simulink library "Tire_MFEval"  (R2026a)
settings: Solver=VariableStepAuto
undefined symbols (not defined in the file): Tire, Visual
libraries: nesl_utility x11, sm_lib x3, mfeval_LIB x1, Tire_Utilities x1, TireBody_Systems x1
Description:
  | Component of Simscape Vehicle Templates Library
  | 
  | Copyright 2018-2024 The MathWorks, Inc.
settings Model: Creator=smiller  LastModifiedBy=andrei

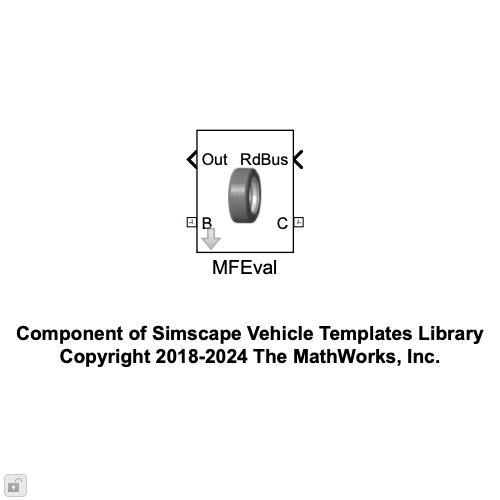
[thumbnail: Simulink's stored preview of the top-level diagram]
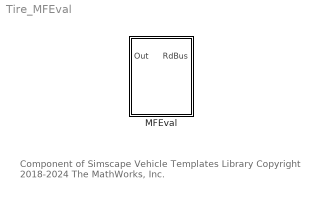
== system Tire_MFEval ==
  note: Component of Simscape Vehicle Templates Library
      | Copyright 2018-2024 The MathWorks, Inc.
  MFEval : Subsystem  VariantControl=MFEval  mask(MFeval Tire){tir_file=Tire.tirFile.Value, tir_side=2 right, tir_dynamics=Tire.Dynamics.Value, tir_mode=Tire.Mode.Value, TireBody=Tire.TireBody, popup_leftRight=Right, clr_tyre=Visual.Tire.clr, opc_tyre=Visual.Tire.opc, clr_rim=Visual.Rim.clrVisual.Rim.clr, opc_rim=Visual.Rim.opc}
      mask prompts: tir_file "TIR File (String variable)"; tir_side "Tyre side     :"; tir_dynamics "Dynamics"; tir_mode "Mode"; TireBody "Tire Body (structure)"; popup_leftRight "Left/Right"
      mask help: Models tire using MFeval tire software.
      mask init:
      | curblk = gcb;
      | tir_file = strrep(tir_file,"''","'");
      | temptirparams = mfeval.readTIR(eval(tir_file));
      | tire_radius = temptirparams.UNLOADED_RADIUS;
      | tire_width  = temptirparams.WIDTH;
      | rim_radius  = temptirparams.RIM_RADIUS;
      | rim_width   = tire_width*0.1;
      | tyre_mass   = temptirparams.MASS1;
      | %if(isnan(tire_mass))
      | %    tire_mass = 15;
      | %end
      | TireStruct = temptirparams;
      | tyre_Ixx   = temptirparams.IXX;
      | tyre_Iyy   = temptirparams.IYY;
      | 
      | tire_kvert  = temptirparams.VERTICAL_STIFFNESS;
      | tire_bvert  = temptirparams.VERTICAL_DAMPING;
      | 
      | %set_param([gcb '/CPI tyre'],'userSide',tir_sie);
      | set_param([gcb '/CPI tyre'],'userDynamics',tir_dynamics);
      | set_param([gcb '/CPI tyre'],'userUseMode',tir_mode);
      | 
      | if(popup_leftRight == 1)
      |     set_param([gcb '/Tire Body'],'popup_leftRight','Left');
      | elseif(popup_leftRight == 2)
      |     set_param([gcb '/Tire Body'],'popup_leftRight','Right');
      | end
      mask TypeOptions tir_side: CPI tyre/userSide
      mask TypeOptions popup_leftRight: Left | Right
      mask TypeOptions clr_tyre: Tire Body/clr_tyre
      mask TypeOptions opc_tyre: Tire Body/opc_tyre
      mask TypeOptions clr_rim: Tire Body/clr_rim
      mask TypeOptions opc_rim: Tire Body/opc_rim
      mask DialogControl cont_tire_mfeval Prompt: Tire
      mask DialogControl cont_vis Prompt: Visualization
      mask DialogControl text_vis_clr Prompt: Color [RGB]
      mask DialogControl text_vis_opc Prompt: Opacity (0-1)
      mask DialogControl text_tyre Prompt: Tyre
      mask DialogControl text_rim Prompt: Rim
      mask Display: image('sm_car_vehicle_tire_mfeval_IMAGE.png');

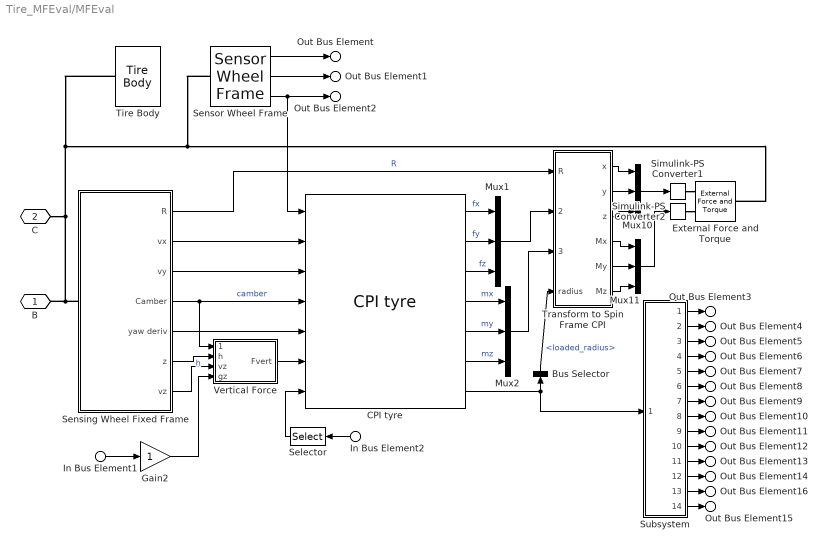
== system Tire_MFEval/MFEval ==
  In Bus Element1 : Inport  PortName=RdBus  Element=gz
  In Bus Element2 : Inport  PortName=RdBus  Element=TyreScaling
  Bus Selector : BusSelector  OutputSignals=loaded_radius
  CPI tyre : mfeval_LIB/CPI tyre  Description=Magic Formula 6.1.2 tyre model including relaxation length and transient calculations  userParameterSource=TireStruct  userSide=2 right  userDynamics=3 non-linear transients  userUseMode=1 combined  enablePressure=off  userPressure=0.5
      settings: SourceProductName=MFeval Library
  External Force and Torque : sm_lib/Forces and Torques/External Force and Torque  EnableForceX=off  EnableForceY=off  EnableForceZ=off  EnableForce=on  ForceResolutionFrame=AttachedFrame  EnableTorqueX=off  EnableTorqueY=off  EnableTorqueZ=off  EnableTorque=on  TorqueResolutionFrame=AttachedFrame
  Gain2 : Gain
  Mux{1..2,10..11} (4 alike) : Mux  Inputs=3
  Selector : Selector  InputPortWidth=7  IndexOptions=Index vector (dialog)  Indices=[1 3]  OutputSizes=1
  Sensing Wheel Fixed Frame : Subsystem
  Sensor Wheel Frame : Tire_Utilities/Sensor Wheel Frame  SystemSampleTime=-1  VariantActivationTime=update diagram  EmptyChoice=off  PassThrough=off  PassThroughVariantControl=(default)  EmptyChoiceVariantControl=(default)  AllowFlexibleInterface=on  Latency=0  AutoFrameSizeCalculation=off
  Simulink-PS Converter1 : nesl_utility/Simulink-PS Converter  PhysicalDomain=network_engine_domain  SubClassName=ps_input  LeftPortType=input  RightPortType=output  PseudoPeriodic=off  Frequencies=[]  NoiseDistribution=none  NoiseParameters=[]  Unit=N  AffineConversion=off  FilteringAndDerivatives=provide  SimscapeFilterOrder=1  InputFilterTimeConstant=0.001  UdotUserProvided=0
  Simulink-PS Converter2 : nesl_utility/Simulink-PS Converter  PhysicalDomain=network_engine_domain  SubClassName=ps_input  LeftPortType=input  RightPortType=output  PseudoPeriodic=off  Frequencies=[]  NoiseDistribution=none  NoiseParameters=[]  Unit=N*m  AffineConversion=off  FilteringAndDerivatives=provide  SimscapeFilterOrder=1  InputFilterTimeConstant=0.001  UdotUserProvided=0
  Subsystem : Subsystem
  Tire Body : TireBody_Systems/Tire Body  LabelModeActiveChoice=Parameterized  popup_leftRight=Left  TireBody=TireBody  VariantLabel=TireBody.class.Value
      settings: AttributesFormatString=%<LabelModeActiveChoice>
  Transform to Spin Frame CPI : Subsystem
  Vertical Force : Subsystem
  B : PMIOPort  Side=Right
  C : PMIOPort  Port=2  Side=Left
  Out Bus Element : Outport  VectorParamsAs1DForOutWhenUnconnected=off  PortName=Out  Element=qxyz
  Out Bus Element1 : Outport  VectorParamsAs1DForOutWhenUnconnected=off  PortName=Out  Element=xyz
  Out Bus Element2 : Outport  VectorParamsAs1DForOutWhenUnconnected=off  PortName=Out  Element=n
  Out Bus Element3 : Outport  VectorParamsAs1DForOutWhenUnconnected=off  PortName=Out  Element=Fx
  Out Bus Element4 : Outport  VectorParamsAs1DForOutWhenUnconnected=off  PortName=Out  Element=Fy
  Out Bus Element5 : Outport  VectorParamsAs1DForOutWhenUnconnected=off  PortName=Out  Element=Fz
  Out Bus Element6 : Outport  VectorParamsAs1DForOutWhenUnconnected=off  PortName=Out  Element=Mx
  Out Bus Element7 : Outport  VectorParamsAs1DForOutWhenUnconnected=off  PortName=Out  Element=My
  Out Bus Element8 : Outport  VectorParamsAs1DForOutWhenUnconnected=off  PortName=Out  Element=Mz
  Out Bus Element9 : Outport  VectorParamsAs1DForOutWhenUnconnected=off  PortName=Out  Element=rSlip
  Out Bus Element10 : Outport  VectorParamsAs1DForOutWhenUnconnected=off  PortName=Out  Element=aSlip
  Out Bus Element11 : Outport  VectorParamsAs1DForOutWhenUnconnected=off  PortName=Out  Element=aCamber
  Out Bus Element12 : Outport  VectorParamsAs1DForOutWhenUnconnected=off  PortName=Out  Element=vx
  Out Bus Element13 : Outport  VectorParamsAs1DForOutWhenUnconnected=off  PortName=Out  Element=rMuX
  Out Bus Element14 : Outport  VectorParamsAs1DForOutWhenUnconnected=off  PortName=Out  Element=rMuY
  Out Bus Element15 : Outport  VectorParamsAs1DForOutWhenUnconnected=off  PortName=Out  Element=r_eff
  Out Bus Element16 : Outport  VectorParamsAs1DForOutWhenUnconnected=off  PortName=Out  Element=r_l
  wires:
  Bus Selector/1 -> Transform to Spin Frame CPI/4(radius)  "<loaded_radius>"
  Sensor Wheel Frame/3 -> CPI tyre/1, Out Bus Element2/1
  Sensor Wheel Frame/2 -> Out Bus Element1/1
  Sensor Wheel Frame/1 -> Out Bus Element/1
  Mux1/1 -> Transform to Spin Frame CPI/2(Fcontact)
  Mux2/1 -> Transform to Spin Frame CPI/3(MContact)
  Mux10/1 -> Simulink-PS Converter1/1
  Transform to Spin Frame CPI/2(y) -> Mux10/2
  Transform to Spin Frame CPI/3(z) -> Mux10/3
  Transform to Spin Frame CPI/5(My) -> Mux11/2
  Transform to Spin Frame CPI/4(Mx) -> Mux11/1
  Transform to Spin Frame CPI/6(Mz) -> Mux11/3
  Transform to Spin Frame CPI/1(x) -> Mux10/1
  Mux11/1 -> Simulink-PS Converter2/1
  Gain2/1 -> Vertical Force/4(gz)
  Sensing Wheel Fixed Frame/7(vz) -> Vertical Force/3(vz)
  Sensing Wheel Fixed Frame/6(z) -> Vertical Force/2(h)  "h"
  Sensing Wheel Fixed Frame/4(Camber) -> Vertical Force/1(camber), CPI tyre/4  "camber"
  Sensing Wheel Fixed Frame/2(vx) -> CPI tyre/2
  CPI tyre/4 -> Mux2/1  "mx"
  CPI tyre/2 -> Mux1/2  "fy"
  CPI tyre/5 -> Mux2/2  "my"
  CPI tyre/6 -> Mux2/3  "mz"
  CPI tyre/3 -> Mux1/3  "fz"
  CPI tyre/1 -> Mux1/1  "fx"
  Vertical Force/1(Fvert) -> CPI tyre/6
  Sensing Wheel Fixed Frame/3(vy) -> CPI tyre/3
  Sensing Wheel Fixed Frame/5(yaw deriv) -> CPI tyre/5
  Sensing Wheel Fixed Frame/1(R) -> Transform to Spin Frame CPI/1(R)  "R"
  In Bus Element1/1 -> Gain2/1
  CPI tyre/7 -> Bus Selector/1, Subsystem/1(In1)
  Subsystem/1(<Fx>) -> Out Bus Element3/1
  Subsystem/2(<Fy>) -> Out Bus Element4/1
  Subsystem/3(<Fz>) -> Out Bus Element5/1
  Subsystem/4(<Mx>) -> Out Bus Element6/1
  Subsystem/5(<My>) -> Out Bus Element7/1
  Subsystem/6(<Mz>) -> Out Bus Element8/1
  Subsystem/7(<longitudinal_slip>) -> Out Bus Element9/1
  Subsystem/8(<side_slip_angle>) -> Out Bus Element10/1
  Subsystem/9(<inclination_angle>) -> Out Bus Element11/1
  Subsystem/10(<Vx>) -> Out Bus Element12/1
  Subsystem/11(<mu_x>) -> Out Bus Element13/1
  Subsystem/12(<mu_y>) -> Out Bus Element14/1
  In Bus Element2/1 -> Selector/1
  Selector/1 -> CPI tyre/7
  Subsystem/13(<r_l>) -> Out Bus Element16/1
  Subsystem/14(<r_eff>) -> Out Bus Element15/1
  connections:
  Simulink-PS Converter1/RConn1 -- External Force and Torque/LConn1
  Simulink-PS Converter2/RConn1 -- External Force and Torque/LConn2
  B/RConn1 -- Sensing Wheel Fixed Frame/LConn1 -- External Force and Torque/RConn1 -- Sensor Wheel Frame/LConn1 -- Tire Body/LConn1 -- C/RConn1

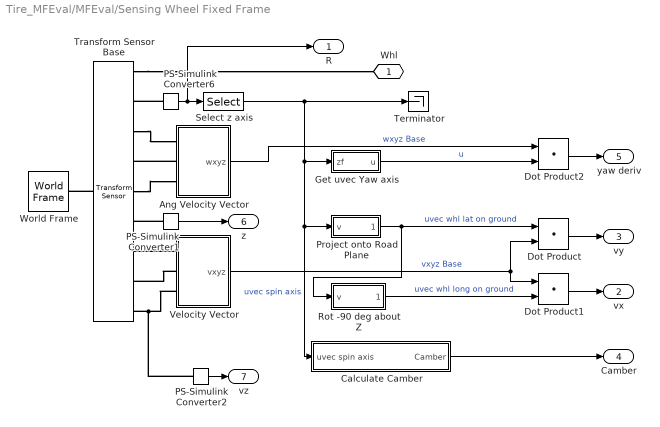
== system Tire_MFEval/MFEval/Sensing Wheel Fixed Frame ==
  Ang Velocity Vector : Subsystem
  Calculate Camber : Subsystem
  Dot Product : DotProduct  OutDataTypeStr=Inherit: Inherit via internal rule
  Dot Product1 : DotProduct  OutDataTypeStr=Inherit: Inherit via internal rule
  Dot Product2 : DotProduct  OutDataTypeStr=Inherit: Inherit via internal rule
  Get uvec Yaw axis : Subsystem
  PS-Simulink Converter1 : nesl_utility/PS-Simulink Converter  PhysicalDomain=network_engine_domain  SubClassName=ps_output  LeftPortType=input  RightPortType=output  PseudoPeriodic=off  Frequencies=[]  VectorFormat=1-D array  Unit=1  AffineConversion=off
  PS-Simulink Converter2 : nesl_utility/PS-Simulink Converter  PhysicalDomain=network_engine_domain  SubClassName=ps_output  LeftPortType=input  RightPortType=output  PseudoPeriodic=off  Frequencies=[]  VectorFormat=1-D array  Unit=1  AffineConversion=off
  PS-Simulink Converter6 : nesl_utility/PS-Simulink Converter  PhysicalDomain=network_engine_domain  SubClassName=ps_output  LeftPortType=input  RightPortType=output  PseudoPeriodic=off  Frequencies=[]  VectorFormat=1-D array  Unit=1  AffineConversion=off
  Project onto Road Plane : Subsystem
  Rot -90 deg about Z : Subsystem
  Select z axis : Selector  NumberOfDimensions=2  InputPortWidth=2  IndexOptions=Index vector (dialog),Index vector (dialog)  Indices=[1 2 3],3  OutputSizes=1,1
  Terminator : Terminator
  Transform Sensor Base : sm_lib/Frames and Transforms/Transform Sensor  MeasurementFrame=Base  RotationSequence=XYX  SenseAngle=off  SenseAxis=off  SenseQ=off  SenseR=on  SenseRotationSequence=off  SenseOmegaX=on  SenseOmegaY=on  SenseOmegaZ=on  SenseOmega=off  SenseQDot=off  SenseRDot=off  SenseRotationSequenceDot=off  SenseAlphaX=off  SenseAlphaY=off  SenseAlphaZ=off  SenseAlpha=off  SenseQDDot=off  SenseRDDot=off  SenseX=off  SenseY=off  SenseZ=on  SenseXYZ=off  SenseRad=off  SenseAzim=off  SenseDist=off  SenseInc=off  SenseXDot=on  SenseYDot=on  SenseZDot=on  SenseXYZDot=off  SenseRadDot=off  SenseAzimDot=off  SenseDistDot=off  SenseIncDot=off  SenseXDDot=off  SenseYDDot=off  SenseZDDot=off  SenseXYZDDot=off  SenseRadDDot=off  SenseAzimDDot=off  SenseDistDDot=off  SenseIncDDot=off
  Velocity Vector : Subsystem
  World Frame : sm_lib/Frames and Transforms/World Frame
  Whl : PMIOPort  Side=Left
  R : Outport  VectorParamsAs1DForOutWhenUnconnected=off
  vx : Outport  Port=2  VectorParamsAs1DForOutWhenUnconnected=off
  vy : Outport  Port=3  VectorParamsAs1DForOutWhenUnconnected=off
  Camber : Outport  Port=4  VectorParamsAs1DForOutWhenUnconnected=off
  yaw deriv : Outport  Port=5  VectorParamsAs1DForOutWhenUnconnected=off
  z : Outport  Port=6  VectorParamsAs1DForOutWhenUnconnected=off
  vz : Outport  Port=7  VectorParamsAs1DForOutWhenUnconnected=off
  wires:
  PS-Simulink Converter2/1 -> vz/1
  PS-Simulink Converter6/1 -> Select z axis/1, R/1
  Select z axis/1 -> Get uvec Yaw axis/1(zf), Calculate Camber/1(uvec spin axis), Project onto Road Plane/1(v), Terminator/1  "uvec spin axis"
  Rot -90 deg about Z/1(v rot -z) -> Dot Product1/2  "uvec whl long on ground"
  Velocity Vector/1(vxyz) -> Dot Product/2, Dot Product1/1  "vxyz Base"
  Get uvec Yaw axis/1(u) -> Dot Product2/2  "u"
  Ang Velocity Vector/1(wxyz) -> Dot Product2/1  "wxyz Base"
  Dot Product2/1 -> yaw deriv/1
  Project onto Road Plane/1(v proj) -> Rot -90 deg about Z/1(v), Dot Product/1  "uvec whl lat on ground"
  Dot Product/1 -> vy/1
  Dot Product1/1 -> vx/1
  PS-Simulink Converter1/1 -> z/1
  Calculate Camber/1(Camber) -> Camber/1
  connections:
  Transform Sensor Base/RConn1 -- Whl/RConn1
  PS-Simulink Converter6/LConn1 -- Transform Sensor Base/RConn2
  Transform Sensor Base/LConn1 -- World Frame/RConn1
  Transform Sensor Base/RConn3 -- Ang Velocity Vector/LConn1
  Ang Velocity Vector/LConn2 -- Transform Sensor Base/RConn4
  Transform Sensor Base/RConn5 -- Ang Velocity Vector/LConn3
  Velocity Vector/LConn1 -- Transform Sensor Base/RConn7
  Velocity Vector/LConn2 -- Transform Sensor Base/RConn8
  PS-Simulink Converter2/LConn1 -- Transform Sensor Base/RConn9 -- Velocity Vector/LConn3
  PS-Simulink Converter1/LConn1 -- Transform Sensor Base/RConn6

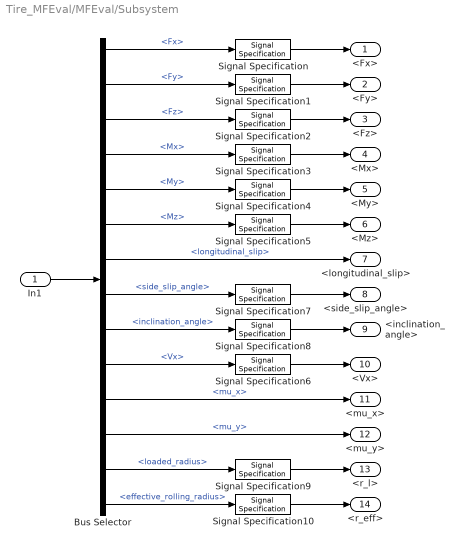
== system Tire_MFEval/MFEval/Subsystem ==
  In1 : Inport
  Bus Selector : BusSelector  OutputSignals=Fx,Fy,Fz,Mx,My,Mz,longitudinal_slip,side_slip_angle,inclination_angle,Vx,mu_x,mu_y,loaded_radius,effective_rolling_radius
  Signal Specification : SignalSpecification  Unit=N
  Signal Specification1 : SignalSpecification  Unit=N
  Signal Specification10 : SignalSpecification  Unit=m
  Signal Specification2 : SignalSpecification  Unit=N
  Signal Specification3 : SignalSpecification  Unit=N*m
  Signal Specification4 : SignalSpecification  Unit=N*m
  Signal Specification5 : SignalSpecification  Unit=N*m
  Signal Specification6 : SignalSpecification  Unit=m/s
  Signal Specification7 : SignalSpecification  Unit=rad
  Signal Specification8 : SignalSpecification  Unit=rad
  Signal Specification9 : SignalSpecification  Unit=m
  <Fx> : Outport  VectorParamsAs1DForOutWhenUnconnected=off
  <Fy> : Outport  Port=2  VectorParamsAs1DForOutWhenUnconnected=off
  <Fz> : Outport  Port=3  VectorParamsAs1DForOutWhenUnconnected=off
  <Mx> : Outport  Port=4  VectorParamsAs1DForOutWhenUnconnected=off
  <My> : Outport  Port=5  VectorParamsAs1DForOutWhenUnconnected=off
  <Mz> : Outport  Port=6  VectorParamsAs1DForOutWhenUnconnected=off
  <longitudinal_slip> : Outport  Port=7  VectorParamsAs1DForOutWhenUnconnected=off
  <side_slip_angle> : Outport  Port=8  VectorParamsAs1DForOutWhenUnconnected=off
  <inclination_angle> : Outport  Port=9  VectorParamsAs1DForOutWhenUnconnected=off
  <Vx> : Outport  Port=10  VectorParamsAs1DForOutWhenUnconnected=off
  <mu_x> : Outport  Port=11  VectorParamsAs1DForOutWhenUnconnected=off
  <mu_y> : Outport  Port=12  VectorParamsAs1DForOutWhenUnconnected=off
  <r_l> : Outport  Port=13  VectorParamsAs1DForOutWhenUnconnected=off
  <r_eff> : Outport  Port=14  VectorParamsAs1DForOutWhenUnconnected=off
  wires:
  Bus Selector/9 -> Signal Specification8/1  "<inclination_angle>"
  Bus Selector/10 -> Signal Specification6/1  "<Vx>"
  Bus Selector/2 -> Signal Specification1/1  "<Fy>"
  Bus Selector/4 -> Signal Specification3/1  "<Mx>"
  Bus Selector/3 -> Signal Specification2/1  "<Fz>"
  Bus Selector/11 -> <mu_x>/1  "<mu_x>"
  Bus Selector/6 -> Signal Specification5/1  "<Mz>"
  Bus Selector/1 -> Signal Specification/1  "<Fx>"
  Bus Selector/8 -> Signal Specification7/1  "<side_slip_angle>"
  Bus Selector/5 -> Signal Specification4/1  "<My>"
  Bus Selector/7 -> <longitudinal_slip>/1  "<longitudinal_slip>"
  Bus Selector/12 -> <mu_y>/1  "<mu_y>"
  In1/1 -> Bus Selector/1
  Signal Specification/1 -> <Fx>/1
  Signal Specification1/1 -> <Fy>/1
  Signal Specification2/1 -> <Fz>/1
  Signal Specification3/1 -> <Mx>/1
  Signal Specification4/1 -> <My>/1
  Signal Specification5/1 -> <Mz>/1
  Signal Specification6/1 -> <Vx>/1
  Signal Specification7/1 -> <side_slip_angle>/1
  Signal Specification8/1 -> <inclination_angle>/1
  Bus Selector/13 -> Signal Specification9/1  "<loaded_radius>"
  Bus Selector/14 -> Signal Specification10/1  "<effective_rolling_radius>"
  Signal Specification9/1 -> <r_l>/1
  Signal Specification10/1 -> <r_eff>/1

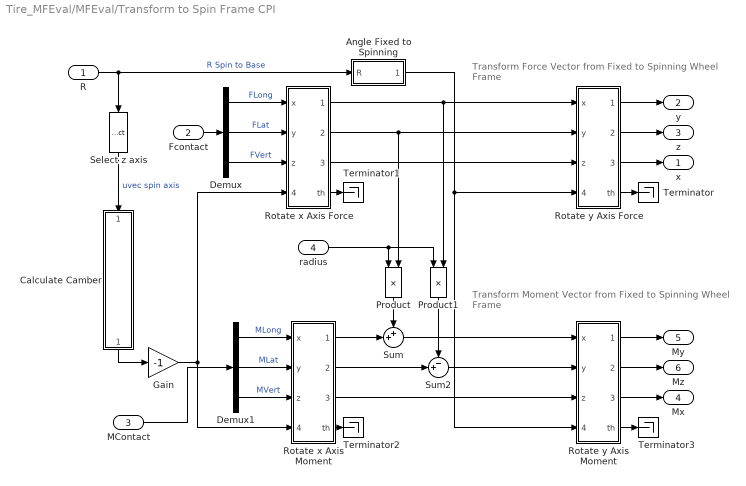
== system Tire_MFEval/MFEval/Transform to Spin Frame CPI ==
  note: Transform Moment Vector from Fixed
      | to Spinning Wheel Frame
  note: Transform Force Vector from Fixed
      | to Spinning Wheel Frame
  R : Inport
  Fcontact : Inport  Port=2
  MContact : Inport  Port=3
  radius : Inport  Port=4
  Angle Fixed to Spinning : Subsystem
  Calculate Camber : Subsystem
  Demux : Demux  Outputs=3
  Demux1 : Demux  Outputs=3
  Gain : Gain  Gain=-1
  Product : Product
  Product1 : Product
  Rotate x Axis Force : Subsystem
  Rotate x Axis Moment : Subsystem
  Rotate y Axis Force : Subsystem
  Rotate y Axis Moment : Subsystem
  Select z axis : Selector  NumberOfDimensions=2  InputPortWidth=2  IndexOptions=Index vector (dialog),Index vector (dialog)  Indices=[1 2 3],3  OutputSizes=1,1
  Sum : Sum  Inputs=++|
  Sum2 : Sum  Inputs=-+|
  Terminator{,1..3} (4 alike) : Terminator
  x : Outport  VectorParamsAs1DForOutWhenUnconnected=off
  y : Outport  Port=2  VectorParamsAs1DForOutWhenUnconnected=off
  z : Outport  Port=3  VectorParamsAs1DForOutWhenUnconnected=off
  Mx : Outport  Port=4  VectorParamsAs1DForOutWhenUnconnected=off
  My : Outport  Port=5  VectorParamsAs1DForOutWhenUnconnected=off
  Mz : Outport  Port=6  VectorParamsAs1DForOutWhenUnconnected=off
  wires:
  R/1 -> Select z axis/1, Angle Fixed to Spinning/1(R)  "R Spin to Base"
  Angle Fixed to Spinning/1(rotang) -> Rotate y Axis Moment/4(theta), Rotate y Axis Force/4(theta)
  Rotate y Axis Moment/1(x rot) -> My/1
  Rotate y Axis Moment/2(y rot) -> Mz/1
  Rotate x Axis Moment/1(x rot) -> Sum/2
  Rotate x Axis Force/1(x rot) -> Product1/2, Rotate y Axis Force/1(x)
  Rotate y Axis Force/1(x rot) -> y/1
  Rotate y Axis Force/2(y rot) -> z/1
  Select z axis/1 -> Calculate Camber/1(uvec spin axis)  "uvec spin axis"
  Demux/1 -> Rotate x Axis Force/1(x)  "FLong"
  Demux/3 -> Rotate x Axis Force/3(z)  "FVert"
  Calculate Camber/1(Camber) -> Gain/1
  Demux1/3 -> Rotate x Axis Moment/3(z)  "MVert"
  Demux1/1 -> Rotate x Axis Moment/1(x)  "MLong"
  Demux1/2 -> Rotate x Axis Moment/2(y)  "MLat"
  Product/1 -> Sum/1
  radius/1 -> Product1/1, Product/1
  Rotate x Axis Force/3(z rot) -> Rotate y Axis Force/3(z)
  Product1/1 -> Sum2/1
  Demux/2 -> Rotate x Axis Force/2(y)  "FLat"
  Rotate x Axis Force/2(y rot) -> Rotate y Axis Force/2(y), Product/2
  Rotate y Axis Force/3(z rot) -> x/1
  Rotate y Axis Force/4(th) -> Terminator/1
  Rotate x Axis Force/4(th) -> Terminator1/1
  Rotate x Axis Moment/2(y rot) -> Sum2/2
  Rotate x Axis Moment/4(th) -> Terminator2/1
  Rotate y Axis Moment/3(z rot) -> Mx/1
  Rotate y Axis Moment/4(th) -> Terminator3/1
  Sum2/1 -> Rotate y Axis Moment/2(y)
  Sum/1 -> Rotate y Axis Moment/1(x)
  Rotate x Axis Moment/3(z rot) -> Rotate y Axis Moment/3(z)
  Gain/1 -> Rotate x Axis Force/4(theta), Rotate x Axis Moment/4(theta)
  Fcontact/1 -> Demux/1
  MContact/1 -> Demux1/1

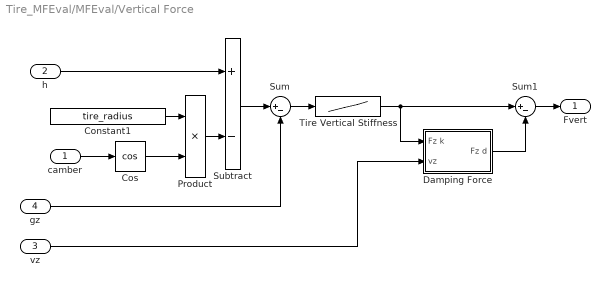
== system Tire_MFEval/MFEval/Vertical Force ==
  camber : Inport
  h : Inport  Port=2
  vz : Inport  Port=3
  gz : Inport  Port=4
  Constant1 : Constant  Value=tire_radius
  Cos : Trigonometry  Operator=cos
  Damping Force : Subsystem
  Product : Product
  Subtract : Sum  Inputs=+-
  Sum : Sum  Inputs=|+-
  Sum1 : Sum  Inputs=|+-
  Tire Vertical Stiffness : Lookup_n-D  NumberOfTableDimensions=1  BreakpointsForDimension1=[-1 0 0.1]  Table=[tire_kvert 0 0]  InternalRulePriority=Speed  RndMeth=Simplest
  Fvert : Outport  VectorParamsAs1DForOutWhenUnconnected=off
  wires:
  h/1 -> Subtract/1
  Sum1/1 -> Fvert/1
  camber/1 -> Cos/1
  gz/1 -> Sum/2
  Cos/1 -> Product/2
  vz/1 -> Damping Force/2(vz)
  Subtract/1 -> Sum/1
  Damping Force/1(Fz d) -> Sum1/2
  Product/1 -> Subtract/2
  Sum/1 -> Tire Vertical Stiffness/1
  Constant1/1 -> Product/1
  Tire Vertical Stiffness/1 -> Damping Force/1(Fz k), Sum1/1

== system Tire_MFEval/MFEval/Sensing Wheel Fixed Frame/Ang Velocity Vector ==
  Mux : Mux  Inputs=3
  PS-Simulink Converter1 : nesl_utility/PS-Simulink Converter  PhysicalDomain=network_engine_domain  SubClassName=ps_output  LeftPortType=input  RightPortType=output  PseudoPeriodic=off  Frequencies=[]  VectorFormat=1-D array  Unit=1  AffineConversion=off
  PS-Simulink Converter2 : nesl_utility/PS-Simulink Converter  PhysicalDomain=network_engine_domain  SubClassName=ps_output  LeftPortType=input  RightPortType=output  PseudoPeriodic=off  Frequencies=[]  VectorFormat=1-D array  Unit=1  AffineConversion=off
  PS-Simulink Converter3 : nesl_utility/PS-Simulink Converter  PhysicalDomain=network_engine_domain  SubClassName=ps_output  LeftPortType=input  RightPortType=output  PseudoPeriodic=off  Frequencies=[]  VectorFormat=1-D array  Unit=rad/s  AffineConversion=off
  Scope : Scope
      settings: ActiveDisplayYMinimum=-5.8089  ActiveDisplayYMaximum=30.87099  DataLoggingVariableName=ScopeData4
  wx : PMIOPort  Side=Left
  wy : PMIOPort  Port=2  Side=Left
  wz : PMIOPort  Port=3  Side=Left
  wxyz : Outport  VectorParamsAs1DForOutWhenUnconnected=off
  wires:
  PS-Simulink Converter1/1 -> Mux/1
  PS-Simulink Converter3/1 -> Mux/3
  PS-Simulink Converter2/1 -> Mux/2
  Mux/1 -> wxyz/1, Scope/1
  connections:
  PS-Simulink Converter2/LConn1 -- wy/RConn1
  wx/RConn1 -- PS-Simulink Converter1/LConn1
  wz/RConn1 -- PS-Simulink Converter3/LConn1

== system Tire_MFEval/MFEval/Sensing Wheel Fixed Frame/Calculate Camber ==
  uvec spin axis : Inport
  Demux : Demux  Outputs=3
  Mux : Mux  Inputs=2
  Trigonometric Function1 : Trigonometry  Operator=atan2
  magnitude : Fcn  Expr=sqrt(u(1)*u(1)+u(2)*u(2))
  Camber : Outport  VectorParamsAs1DForOutWhenUnconnected=off
  wires:
  Demux/1 -> Mux/1
  uvec spin axis/1 -> Demux/1
  Trigonometric Function1/1 -> Camber/1
  Demux/3 -> Trigonometric Function1/1
  Mux/1 -> magnitude/1
  magnitude/1 -> Trigonometric Function1/2
  Demux/2 -> Mux/2

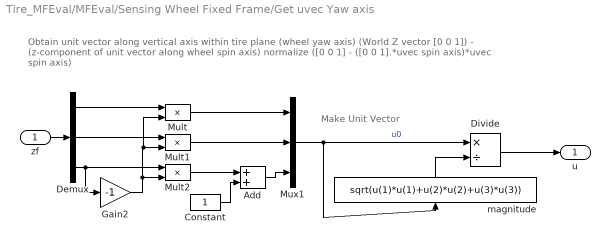
== system Tire_MFEval/MFEval/Sensing Wheel Fixed Frame/Get uvec Yaw axis ==
  note: Make Unit Vector
  note: Obtain unit vector along vertical axis within tire plane (wheel yaw axis)
      | (World Z vector [0 0 1])  -  (z-component of unit vector along wheel spin axis)
      | normalize ([0 0 1] - ([0 0 1].*uvec spin axis)*uvec spin axis)
  zf : Inport
  Add : Sum
  Constant : Constant
  Demux : Demux  Outputs=3
  Divide : Product  Inputs=*/
  Gain2 : Gain  Gain=-1
  Mult : Product  Inputs=**
  Mult1 : Product  Inputs=**
  Mult2 : Product  Inputs=**
  Mux1 : Mux  Inputs=3
  magnitude : Fcn  Expr=sqrt(u(1)*u(1)+u(2)*u(2)+u(3)*u(3))
  u : Outport  VectorParamsAs1DForOutWhenUnconnected=off
  wires:
  Add/1 -> Mux1/3
  Demux/2 -> Mult1/1
  Mux1/1 -> magnitude/1, Divide/1  "u0"
  Mult2/1 -> Add/1
  Demux/1 -> Mult/1
  zf/1 -> Demux/1
  Demux/3 -> Gain2/1, Mult2/1
  Gain2/1 -> Mult2/2, Mult1/2, Mult/2
  Mult1/1 -> Mux1/2
  Mult/1 -> Mux1/1
  Constant/1 -> Add/2
  Divide/1 -> u/1
  magnitude/1 -> Divide/2

== system Tire_MFEval/MFEval/Sensing Wheel Fixed Frame/Project onto Road Plane ==
  note: Normalize to create a unit vector
  note: Create unit vector in lateral direction from wheel on ground plane.
      |
      | This computation projects input vector v (along the wheel spin axis) onto the plane normal to the z axis.
  v : Inport
  Constant : Constant  Value=0
  Demux : Demux  Outputs=3
  Divide : Product  Inputs=*/
  Mux1 : Mux  Inputs=3
  Terminator : Terminator
  magnitude : Fcn  Expr=sqrt(u(1)*u(1)+u(2)*u(2))
  v proj : Outport  VectorParamsAs1DForOutWhenUnconnected=off
  wires:
  Mux1/1 -> Divide/1, magnitude/1
  Demux/2 -> Mux1/2
  Demux/1 -> Mux1/1
  Constant/1 -> Mux1/3
  Demux/3 -> Terminator/1
  v/1 -> Demux/1
  Divide/1 -> v proj/1
  magnitude/1 -> Divide/2

== system Tire_MFEval/MFEval/Sensing Wheel Fixed Frame/Rot -90 deg about Z ==
  v : Inport
  Demux : Demux  Outputs=3
  Gain : Gain  Gain=-1
  Mux1 : Mux  Inputs=3
  v rot -z : Outport  VectorParamsAs1DForOutWhenUnconnected=off
  wires:
  Demux/1 -> Gain/1
  Mux1/1 -> v rot -z/1
  Demux/3 -> Mux1/3
  Gain/1 -> Mux1/2
  Demux/2 -> Mux1/1
  v/1 -> Demux/1

== system Tire_MFEval/MFEval/Sensing Wheel Fixed Frame/Velocity Vector ==
  Mux : Mux  Inputs=3
  PS-Simulink Converter1 : nesl_utility/PS-Simulink Converter  PhysicalDomain=network_engine_domain  SubClassName=ps_output  LeftPortType=input  RightPortType=output  PseudoPeriodic=off  Frequencies=[]  VectorFormat=1-D array  Unit=1  AffineConversion=off
  PS-Simulink Converter2 : nesl_utility/PS-Simulink Converter  PhysicalDomain=network_engine_domain  SubClassName=ps_output  LeftPortType=input  RightPortType=output  PseudoPeriodic=off  Frequencies=[]  VectorFormat=1-D array  Unit=1  AffineConversion=off
  PS-Simulink Converter3 : nesl_utility/PS-Simulink Converter  PhysicalDomain=network_engine_domain  SubClassName=ps_output  LeftPortType=input  RightPortType=output  PseudoPeriodic=off  Frequencies=[]  VectorFormat=1-D array  Unit=1  AffineConversion=off
  vx : PMIOPort  Side=Left
  vy : PMIOPort  Port=2  Side=Left
  vz : PMIOPort  Port=3  Side=Left
  vxyz : Outport  VectorParamsAs1DForOutWhenUnconnected=off
  wires:
  PS-Simulink Converter1/1 -> Mux/1
  PS-Simulink Converter3/1 -> Mux/3
  PS-Simulink Converter2/1 -> Mux/2
  Mux/1 -> vxyz/1
  connections:
  PS-Simulink Converter2/LConn1 -- vy/RConn1
  vx/RConn1 -- PS-Simulink Converter1/LConn1
  vz/RConn1 -- PS-Simulink Converter3/LConn1

== system Tire_MFEval/MFEval/Transform to Spin Frame CPI/Angle Fixed to Spinning ==
  R : Inport
  Atan2 : Trigonometry  Operator=atan2
  Demux1 : Demux  Outputs=3
  Get uvec Yaw axis : Subsystem
  Multiply : Product  Inputs=**  Multiplication=Matrix(*)
  Select z axis : Selector  NumberOfDimensions=2  InputPortWidth=2  IndexOptions=Index vector (dialog),Index vector (dialog)  Indices=[1 2 3],3  OutputSizes=1,1
  Terminator : Terminator
  Transpose : Math  Operator=transpose  SignedPower=on
  rotang : Outport  VectorParamsAs1DForOutWhenUnconnected=off
  wires:
  Demux1/2 -> Atan2/1
  Get uvec Yaw axis/1(u) -> Multiply/2  "Yaw vec Base"
  Demux1/1 -> Atan2/2
  Demux1/3 -> Terminator/1
  Select z axis/1 -> Get uvec Yaw axis/1(zf)  "uvec spin axis"
  R/1 -> Select z axis/1, Transpose/1
  Atan2/1 -> rotang/1
  Multiply/1 -> Demux1/1  "yaw vec spin frame"
  Transpose/1 -> Multiply/1  "R Base 2 Spin Frame"

== system Tire_MFEval/MFEval/Transform to Spin Frame CPI/Calculate Camber ==
  uvec spin axis : Inport
  Demux : Demux  Outputs=3
  Mux : Mux  Inputs=2
  Trigonometric Function1 : Trigonometry  Operator=atan2
  magnitude : Fcn  Expr=sqrt(u(1)*u(1)+u(2)*u(2))
  Camber : Outport  VectorParamsAs1DForOutWhenUnconnected=off
  wires:
  Demux/2 -> Mux/2
  magnitude/1 -> Trigonometric Function1/2
  Mux/1 -> magnitude/1
  Demux/3 -> Trigonometric Function1/1
  Trigonometric Function1/1 -> Camber/1
  uvec spin axis/1 -> Demux/1
  Demux/1 -> Mux/1

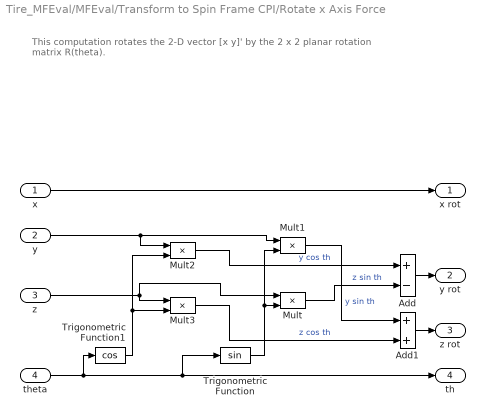
== system Tire_MFEval/MFEval/Transform to Spin Frame CPI/Rotate x Axis Force ==
  note: This computation rotates the 2-D vector [x y]' by the 2 x 2
      | planar rotation matrix R(theta).
  x : Inport
  y : Inport  Port=2
  z : Inport  Port=3
  theta : Inport  Port=4
  Add : Sum  Inputs=+-
  Add1 : Sum
  Mult{,1..3} (4 alike) : Product  Inputs=**
  Trigonometric Function : Trigonometry
  Trigonometric Function1 : Trigonometry  Operator=cos
  x rot : Outport  VectorParamsAs1DForOutWhenUnconnected=off
  y rot : Outport  Port=2  VectorParamsAs1DForOutWhenUnconnected=off
  z rot : Outport  Port=3  VectorParamsAs1DForOutWhenUnconnected=off
  th : Outport  Port=4  VectorParamsAs1DForOutWhenUnconnected=off
  wires:
  theta/1 -> th/1, Trigonometric Function/1, Trigonometric Function1/1
  y/1 -> Mult1/1, Mult2/1
  z/1 -> Mult3/1, Mult/1
  Trigonometric Function1/1 -> Mult2/2, Mult3/2
  Trigonometric Function/1 -> Mult1/2, Mult/2
  Mult2/1 -> Add/1  "y cos th"
  Add/1 -> y rot/1
  Mult3/1 -> Add1/2  "z cos th"
  Add1/1 -> z rot/1
  Mult/1 -> Add/2  "z sin th"
  Mult1/1 -> Add1/1  "y sin th"
  x/1 -> x rot/1

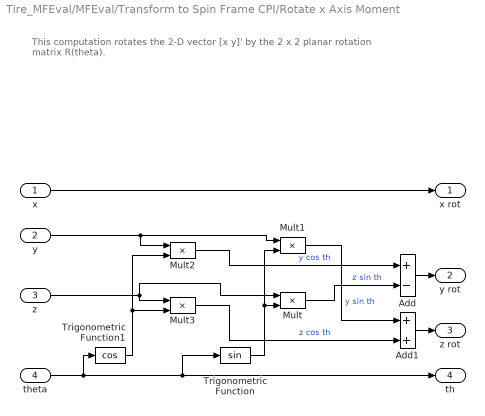
== system Tire_MFEval/MFEval/Transform to Spin Frame CPI/Rotate x Axis Moment ==
  note: This computation rotates the 2-D vector [x y]' by the 2 x 2
      | planar rotation matrix R(theta).
  x : Inport
  y : Inport  Port=2
  z : Inport  Port=3
  theta : Inport  Port=4
  Add : Sum  Inputs=+-
  Add1 : Sum
  Mult{,1..3} (4 alike) : Product  Inputs=**
  Trigonometric Function : Trigonometry
  Trigonometric Function1 : Trigonometry  Operator=cos
  x rot : Outport  VectorParamsAs1DForOutWhenUnconnected=off
  y rot : Outport  Port=2  VectorParamsAs1DForOutWhenUnconnected=off
  z rot : Outport  Port=3  VectorParamsAs1DForOutWhenUnconnected=off
  th : Outport  Port=4  VectorParamsAs1DForOutWhenUnconnected=off
  wires:
  x/1 -> x rot/1
  Mult1/1 -> Add1/1  "y sin th"
  Mult/1 -> Add/2  "z sin th"
  Add1/1 -> z rot/1
  Mult3/1 -> Add1/2  "z cos th"
  Add/1 -> y rot/1
  Mult2/1 -> Add/1  "y cos th"
  Trigonometric Function/1 -> Mult/2, Mult1/2
  Trigonometric Function1/1 -> Mult3/2, Mult2/2
  z/1 -> Mult/1, Mult3/1
  y/1 -> Mult2/1, Mult1/1
  theta/1 -> Trigonometric Function1/1, Trigonometric Function/1, th/1

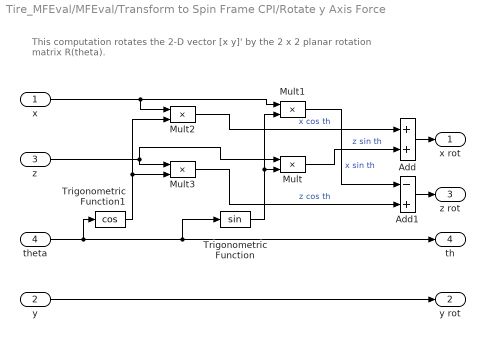
== system Tire_MFEval/MFEval/Transform to Spin Frame CPI/Rotate y Axis Force ==
  note: This computation rotates the 2-D vector [x y]' by the 2 x 2
      | planar rotation matrix R(theta).
  x : Inport
  y : Inport  Port=2
  z : Inport  Port=3
  theta : Inport  Port=4
  Add : Sum
  Add1 : Sum  Inputs=-+
  Mult{,1..3} (4 alike) : Product  Inputs=**
  Trigonometric Function : Trigonometry
  Trigonometric Function1 : Trigonometry  Operator=cos
  x rot : Outport  VectorParamsAs1DForOutWhenUnconnected=off
  y rot : Outport  Port=2  VectorParamsAs1DForOutWhenUnconnected=off
  z rot : Outport  Port=3  VectorParamsAs1DForOutWhenUnconnected=off
  th : Outport  Port=4  VectorParamsAs1DForOutWhenUnconnected=off
  wires:
  Mult1/1 -> Add1/1  "x sin th"
  Mult/1 -> Add/2  "z sin th"
  Add1/1 -> z rot/1
  Mult3/1 -> Add1/2  "z cos th"
  Add/1 -> x rot/1
  Mult2/1 -> Add/1  "x cos th"
  Trigonometric Function/1 -> Mult/2, Mult1/2
  Trigonometric Function1/1 -> Mult3/2, Mult2/2
  z/1 -> Mult/1, Mult3/1
  x/1 -> Mult2/1, Mult1/1
  theta/1 -> Trigonometric Function1/1, th/1, Trigonometric Function/1
  y/1 -> y rot/1

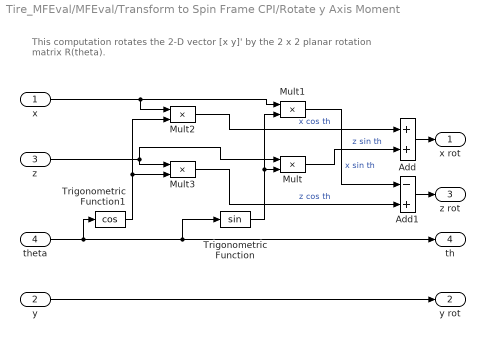
== system Tire_MFEval/MFEval/Transform to Spin Frame CPI/Rotate y Axis Moment ==
  note: This computation rotates the 2-D vector [x y]' by the 2 x 2
      | planar rotation matrix R(theta).
  x : Inport
  y : Inport  Port=2
  z : Inport  Port=3
  theta : Inport  Port=4
  Add : Sum
  Add1 : Sum  Inputs=-+
  Mult{,1..3} (4 alike) : Product  Inputs=**
  Trigonometric Function : Trigonometry
  Trigonometric Function1 : Trigonometry  Operator=cos
  x rot : Outport  VectorParamsAs1DForOutWhenUnconnected=off
  y rot : Outport  Port=2  VectorParamsAs1DForOutWhenUnconnected=off
  z rot : Outport  Port=3  VectorParamsAs1DForOutWhenUnconnected=off
  th : Outport  Port=4  VectorParamsAs1DForOutWhenUnconnected=off
  wires:
  y/1 -> y rot/1
  theta/1 -> Trigonometric Function/1, th/1, Trigonometric Function1/1
  x/1 -> Mult1/1, Mult2/1
  z/1 -> Mult3/1, Mult/1
  Trigonometric Function1/1 -> Mult2/2, Mult3/2
  Trigonometric Function/1 -> Mult1/2, Mult/2
  Mult2/1 -> Add/1  "x cos th"
  Add/1 -> x rot/1
  Mult3/1 -> Add1/2  "z cos th"
  Add1/1 -> z rot/1
  Mult/1 -> Add/2  "z sin th"
  Mult1/1 -> Add1/1  "x sin th"

== system Tire_MFEval/MFEval/Vertical Force/Damping Force ==
  note: Apply damping only when stiffness force >0
  Fz k : Inport
  vz : Inport  Port=2
  Constant : Constant  Value=0
  Constant1 : Constant  Value=tire_bvert
  Product : Product
  Switch : Switch  Criteria=u2 > Threshold  ZeroCross=off  SaturateOnIntegerOverflow=off  InputSameDT=off
  Fz d : Outport  VectorParamsAs1DForOutWhenUnconnected=off
  wires:
  Constant1/1 -> Product/2
  Constant/1 -> Switch/3
  Switch/1 -> Fz d/1
  Fz k/1 -> Switch/2
  Product/1 -> Switch/1
  vz/1 -> Product/1

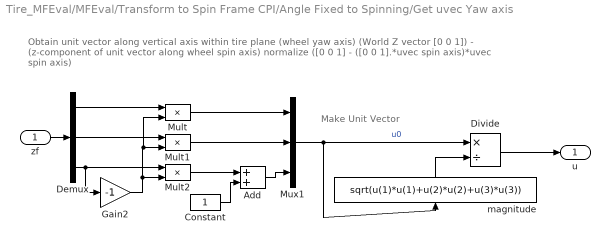
== system Tire_MFEval/MFEval/Transform to Spin Frame CPI/Angle Fixed to Spinning/Get uvec Yaw axis ==
  note: Obtain unit vector along vertical axis within tire plane (wheel yaw axis)
      | (World Z vector [0 0 1])  -  (z-component of unit vector along wheel spin axis)
      | normalize ([0 0 1] - ([0 0 1].*uvec spin axis)*uvec spin axis)
  note: Make Unit Vector
  zf : Inport
  Add : Sum
  Constant : Constant
  Demux : Demux  Outputs=3
  Divide : Product  Inputs=*/
  Gain2 : Gain  Gain=-1
  Mult : Product  Inputs=**
  Mult1 : Product  Inputs=**
  Mult2 : Product  Inputs=**
  Mux1 : Mux  Inputs=3
  magnitude : Fcn  Expr=sqrt(u(1)*u(1)+u(2)*u(2)+u(3)*u(3))
  u : Outport  VectorParamsAs1DForOutWhenUnconnected=off
  wires:
  magnitude/1 -> Divide/2
  Divide/1 -> u/1
  Constant/1 -> Add/2
  Mult/1 -> Mux1/1
  Mult1/1 -> Mux1/2
  Gain2/1 -> Mult/2, Mult1/2, Mult2/2
  Demux/3 -> Mult2/1, Gain2/1
  zf/1 -> Demux/1
  Demux/1 -> Mult/1
  Mult2/1 -> Add/1
  Mux1/1 -> Divide/1, magnitude/1  "u0"
  Demux/2 -> Mult1/1
  Add/1 -> Mux1/3
